simulink model "sfGetStartedFunction"  (R2025b)
settings: Solver=VariableStepAuto  StartTime=0.0  StopTime=200  RelTol=1e-3
settings Model: Creator=The MathWorks, Inc.  LastModifiedBy=The MathWorks, Inc.

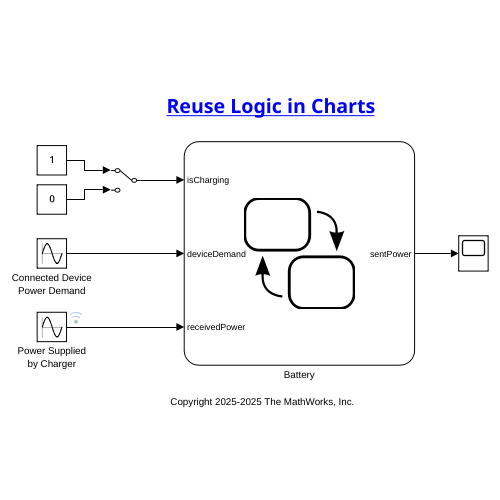
[thumbnail: Simulink's stored preview of the top-level diagram]
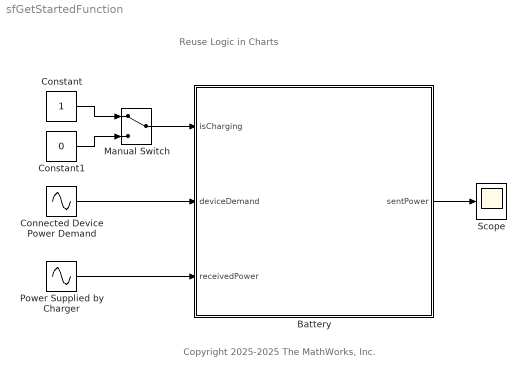
== system sfGetStartedFunction ==
  note: Copyright 2025-2025 The MathWorks, Inc.
  note: Reuse Logic in Charts
  Battery : Stateflow chart  TreatAsAtomicUnit=on
  Connected Device Power Demand : Sin  Amplitude=2.5  Bias=2.5  Phase=-pi/4  SampleTime=0
  Constant : Constant
  Constant1 : Constant  Value=0
  Manual Switch : ManualSwitch
  Power Supplied by Charger : Sin  Amplitude=6  Frequency=0.066  SampleTime=0
  Scope : Scope
      settings: ActiveDisplayYMinimum=-0.43749999999999989  ActiveDisplayYMaximum=3.9375
  wires:
  Manual Switch/1 -> Battery/1(isCharging)
  Constant/1 -> Manual Switch/1
  Constant1/1 -> Manual Switch/2
  Battery/1(sentPower) -> Scope/1
  Connected Device Power Demand/1 -> Battery/2(deviceDemand)
  Power Supplied by Charger/1 -> Battery/3(receivedPower)

== stateflow chart sfGetStartedFunction/Battery ==
  state MainBattery [parallel]
    settings: executionOrder=1
    state Charge
      entry:
      sentPower=0;
      send(toggleOff,EmergencyBattery);
      state FastCharge
        during:
        mainCharge=mainCharge+4;
      state SlowCharge
        during:
        mainCharge=mainCharge+1;
      state Full
      (default) -> FastCharge
      FastCharge -> SlowCharge : [mainCharge>80]
      SlowCharge -> Full : [mainCharge>=100]
    state Discharge
      state Powered
        MainBattery.Discharge.Powered -> (junction 78) [order 1]
        (junction 78) -> (junction 96) [order 1] : [deviceDemand>maxPower]
        (junction 78) -> (junction 94) [order 2] : {sentPower=deviceDemand;}
        (junction 96) -> (junction 95) : {sentPower=maxPower;}
        (junction 95) -> (junction 94)
        (junction 94) -> (junction 90) : {mainCharge=mainCharge-sentPower;}
      state Empty
        entry:
        sentPower=0;
        send(toggleOn,EmergencyBattery);
      (default) -> MainBattery.Discharge.Powered
      MainBattery.Discharge.Powered -> MainBattery.Discharge.Empty [order 1] : [mainCharge<=3]
    (default) -> Charge
    Charge -> MainBattery.Discharge : [~isCharging]
    MainBattery.Discharge -> Charge : [isCharging]
  state EmergencyBattery [parallel]
    settings: executionOrder=2
    state Discharge
      state Powered
        during:
        emergencyCharge=emergencyCharge-0.01;
      state Empty
      (default) -> EmergencyBattery.Discharge.Powered
      EmergencyBattery.Discharge.Powered -> EmergencyBattery.Discharge.Empty : [emergencyCharge<=0.01]
    state Standby
    (default) -> Standby
    Standby -> EmergencyBattery.Discharge : toggleOn
    EmergencyBattery.Discharge -> Standby : toggleOff
  data: isCharging input size=1; sentPower output size=1; mainCharge local size=1 =0; deviceDemand input size=1; maxPower local size=1 =3.5; emergencyCharge local =100; receivedPower input
  events: toggleOff local FUNCTION_CALL_EVENT; toggleOn local FUNCTION_CALL_EVENT
